simulink model "PMLSM_MIL_Library_Sim"  (R2023b)
settings: Solver=FixedStepDiscrete  StartTime=0.0  StopTime=1.5  FixedStep=1e-4  RelTol=1e-3
values from neighbouring files (symbols this model uses):
  PMLSM_grating_resolution_mm = 0.0001    [init_PMLSM_plant_params.m]
  PMLSM_Kf_N_per_A = PMLSM_Kf_peak_N_per_Apeak    [init_PMLSM_plant_params.m]
  PMLSM_Ld_H = Ld    (= 0.001745)    [PMSLM_Init_Params_MBDL4.m]    (also in init_PMLSM_plant_params.m)
  PMLSM_Lq_H = Lq    (= 0.001745)    [PMSLM_Init_Params_MBDL4.m]    (also in init_PMLSM_plant_params.m)
  PMLSM_mass_kg = PMLSM_M_kg    (= 0.91)    [init_PMLSM_plant_params.m]
  PMLSM_psi_f_Wb = flux    (= 0.141)    [PMSLM_Init_Params_MBDL4.m]    (also in init_PMLSM_plant_params.m)
  PMLSM_pwm_period_counts = 7500    [init_PMLSM_plant_params.m]
  PMLSM_Rs_ohm = Rs    (= 2.37)    [PMSLM_Init_Params_MBDL4.m]    (also in init_PMLSM_plant_params.m)
  PMLSM_sensor_delay_samples = 50    [init_PMLSM_plant_params.m]
  PMLSM_tau_e_mm = PMLSM_tau_NN_mm    (= 60)    [init_PMLSM_plant_params.m]
  PMLSM_theta_offset_rad = 0    [init_PMLSM_plant_params.m]
  PMLSM_Ts_s = 1e-4    (= 0.0001)    [init_PMLSM_plant_params.m]
  PMLSM_vdc_V = 48    [init_PMLSM_plant_params.m]
  PMLSM_viscous_N_per_mps = PMLSM_Bv_N_per_mps    (= 0)    [init_PMLSM_plant_params.m]
undefined symbols (not defined in the file or in its folder): DiscIntNeverNeededParam
settings Model: Creator=lww  LastModifiedBy=lww

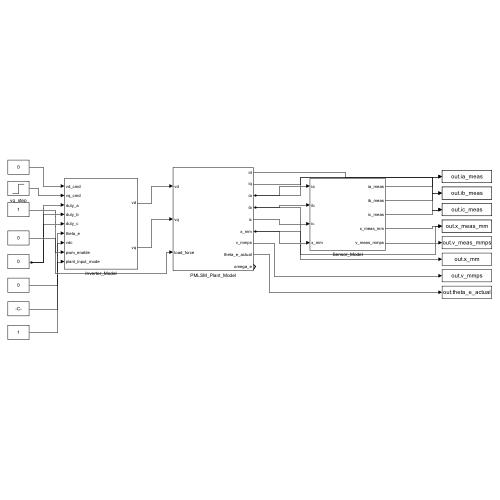
[thumbnail: Simulink's stored preview of the top-level diagram]
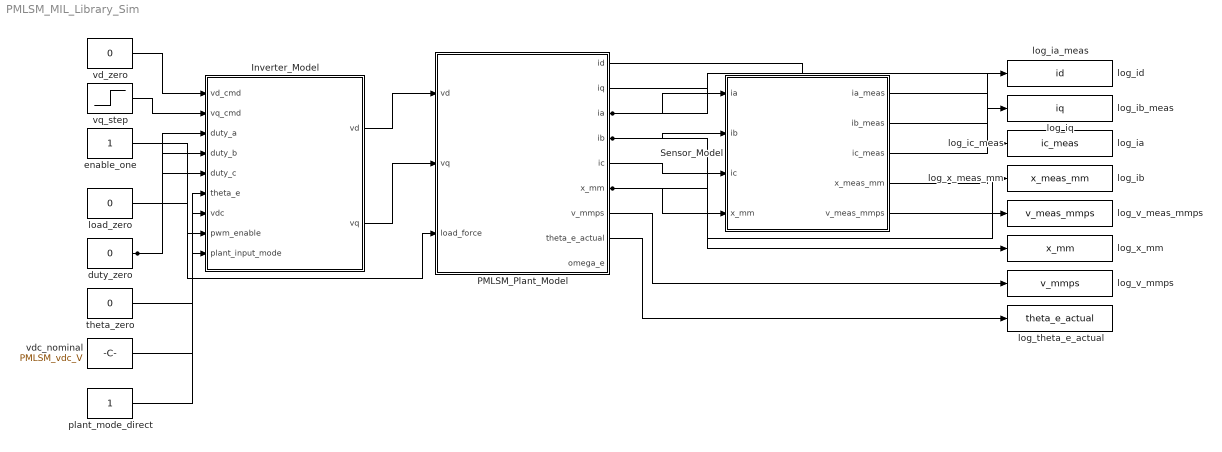
== system PMLSM_MIL_Library_Sim ==
  Inverter_Model : Subsystem
  PMLSM_Plant_Model : Subsystem
  Sensor_Model : Subsystem
  duty_zero : Constant  Value=0
  enable_one : Constant
  load_zero : Constant  Value=0
  log_ia : ToWorkspace  VariableName=ia  SaveFormat=Timeseries  SampleTime=-1
  log_ia_meas : ToWorkspace  VariableName=ia_meas  SaveFormat=Timeseries  SampleTime=-1
  log_ib : ToWorkspace  VariableName=ib  SaveFormat=Timeseries  SampleTime=-1
  log_ib_meas : ToWorkspace  VariableName=ib_meas  SaveFormat=Timeseries  SampleTime=-1
  log_ic_meas : ToWorkspace  VariableName=ic_meas  SaveFormat=Timeseries  SampleTime=-1
  log_id : ToWorkspace  VariableName=id  SaveFormat=Timeseries  SampleTime=-1
  log_iq : ToWorkspace  VariableName=iq  SaveFormat=Timeseries  SampleTime=-1
  log_theta_e_actual : ToWorkspace  VariableName=theta_e_actual  SaveFormat=Timeseries  SampleTime=-1
  log_v_meas_mmps : ToWorkspace  VariableName=v_meas_mmps  SaveFormat=Timeseries  SampleTime=-1
  log_v_mmps : ToWorkspace  VariableName=v_mmps  SaveFormat=Timeseries  SampleTime=-1
  log_x_meas_mm : ToWorkspace  VariableName=x_meas_mm  SaveFormat=Timeseries  SampleTime=-1
  log_x_mm : ToWorkspace  VariableName=x_mm  SaveFormat=Timeseries  SampleTime=-1
  plant_mode_direct : Constant
  theta_zero : Constant  Value=0
  vd_zero : Constant  Value=0
  vdc_nominal : Constant  Value=PMLSM_vdc_V
  vq_step : Step  Time=0.05  After=0.8  SampleTime=0
  wires:
  vd_zero/1 -> Inverter_Model/1(vd_cmd)
  vq_step/1 -> Inverter_Model/2(vq_cmd)
  duty_zero/1 -> Inverter_Model/3(duty_a), Inverter_Model/4(duty_b), Inverter_Model/5(duty_c)
  theta_zero/1 -> Inverter_Model/6(theta_e)
  vdc_nominal/1 -> Inverter_Model/7(vdc)
  enable_one/1 -> Inverter_Model/8(pwm_enable)
  plant_mode_direct/1 -> Inverter_Model/9(plant_input_mode)
  Inverter_Model/1(vd) -> PMLSM_Plant_Model/1(vd)
  Inverter_Model/2(vq) -> PMLSM_Plant_Model/2(vq)
  load_zero/1 -> PMLSM_Plant_Model/3(load_force)
  PMLSM_Plant_Model/3(ia) -> Sensor_Model/1(ia), log_ia/1
  PMLSM_Plant_Model/4(ib) -> Sensor_Model/2(ib), log_ib/1
  PMLSM_Plant_Model/5(ic) -> Sensor_Model/3(ic)
  PMLSM_Plant_Model/6(x_mm) -> Sensor_Model/4(x_mm), log_x_mm/1
  PMLSM_Plant_Model/1(id) -> log_id/1
  PMLSM_Plant_Model/2(iq) -> log_iq/1
  PMLSM_Plant_Model/7(v_mmps) -> log_v_mmps/1
  PMLSM_Plant_Model/8(theta_e_actual) -> log_theta_e_actual/1
  Sensor_Model/1(ia_meas) -> log_ia_meas/1
  Sensor_Model/2(ib_meas) -> log_ib_meas/1
  Sensor_Model/3(ic_meas) -> log_ic_meas/1
  Sensor_Model/4(x_meas_mm) -> log_x_meas_mm/1
  Sensor_Model/5(v_meas_mmps) -> log_v_meas_mmps/1

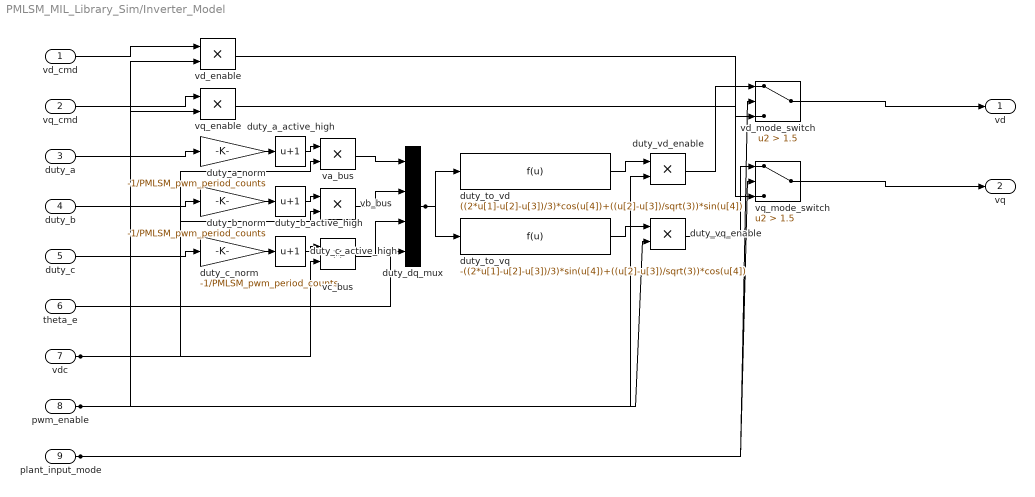
== system PMLSM_MIL_Library_Sim/Inverter_Model ==
  vd_cmd : Inport
  vq_cmd : Inport  Port=2
  duty_a : Inport  Port=3
  duty_b : Inport  Port=4
  duty_c : Inport  Port=5
  theta_e : Inport  Port=6
  vdc : Inport  Port=7
  pwm_enable : Inport  Port=8
  plant_input_mode : Inport  Port=9
  duty_a_active_high : Bias  Bias=1  SaturateOnIntegerOverflow=off
  duty_a_norm : Gain  Gain=-1/PMLSM_pwm_period_counts
  duty_b_active_high : Bias  Bias=1  SaturateOnIntegerOverflow=off
  duty_b_norm : Gain  Gain=-1/PMLSM_pwm_period_counts
  duty_c_active_high : Bias  Bias=1  SaturateOnIntegerOverflow=off
  duty_c_norm : Gain  Gain=-1/PMLSM_pwm_period_counts
  duty_dq_mux : Mux
  duty_to_vd : Fcn  Expr=((2*u[1]-u[2]-u[3])/3)*cos(u[4])+((u[2]-u[3])/sqrt(3))*sin(u[4])
  duty_to_vq : Fcn  Expr=-((2*u[1]-u[2]-u[3])/3)*sin(u[4])+((u[2]-u[3])/sqrt(3))*cos(u[4])
  duty_vd_enable : Product
  duty_vq_enable : Product
  va_bus : Product
  vb_bus : Product
  vc_bus : Product
  vd_enable : Product
  vd_mode_switch : Switch  Criteria=u2 > Threshold  Threshold=1.5  SaturateOnIntegerOverflow=off  InputSameDT=off
  vq_enable : Product
  vq_mode_switch : Switch  Criteria=u2 > Threshold  Threshold=1.5  SaturateOnIntegerOverflow=off  InputSameDT=off
  vd : Outport
  vq : Outport  Port=2
  wires:
  ? -> ?
  vd_cmd/1 -> vd_enable/1
  pwm_enable/1 -> vd_enable/2, vq_enable/2, duty_vd_enable/2, duty_vq_enable/2
  vq_cmd/1 -> vq_enable/1
  duty_a/1 -> duty_a_norm/1
  duty_b/1 -> duty_b_norm/1
  duty_c/1 -> duty_c_norm/1
  duty_a_norm/1 -> duty_a_active_high/1
  duty_b_norm/1 -> duty_b_active_high/1
  duty_c_norm/1 -> duty_c_active_high/1
  duty_a_active_high/1 -> va_bus/1
  duty_b_active_high/1 -> vb_bus/1
  duty_c_active_high/1 -> vc_bus/1
  vdc/1 -> va_bus/2, vb_bus/2, vc_bus/2
  va_bus/1 -> duty_dq_mux/1
  vb_bus/1 -> duty_dq_mux/2
  vc_bus/1 -> duty_dq_mux/3
  theta_e/1 -> duty_dq_mux/4
  duty_dq_mux/1 -> duty_to_vd/1, duty_to_vq/1
  duty_to_vd/1 -> duty_vd_enable/1
  duty_to_vq/1 -> duty_vq_enable/1
  duty_vd_enable/1 -> vd_mode_switch/1
  plant_input_mode/1 -> vd_mode_switch/2, vq_mode_switch/2
  vd_enable/1 -> vd_mode_switch/3
  duty_vq_enable/1 -> vq_mode_switch/1
  vq_enable/1 -> vq_mode_switch/3
  vd_mode_switch/1 -> vd/1
  vq_mode_switch/1 -> vq/1

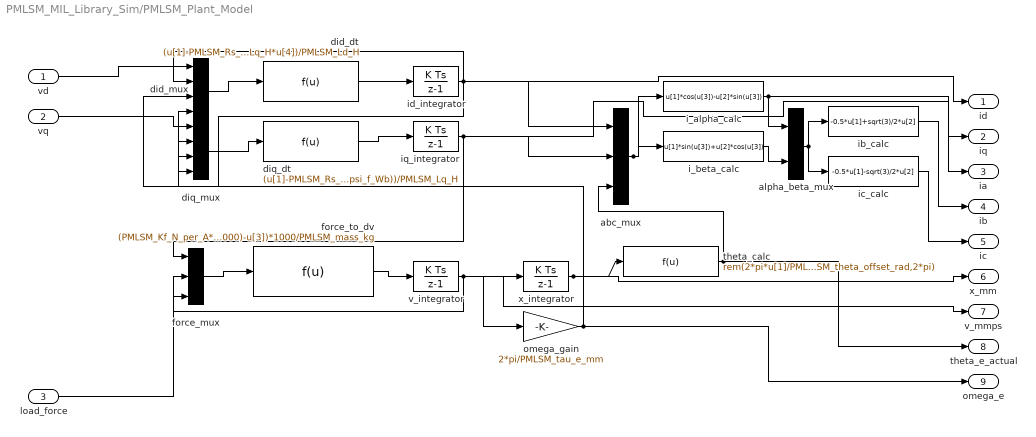
== system PMLSM_MIL_Library_Sim/PMLSM_Plant_Model ==
  vd : Inport
  vq : Inport  Port=2
  load_force : Inport  Port=3
  abc_mux : Mux  Inputs=3
  alpha_beta_mux : Mux  Inputs=2
  did_dt : Fcn  Expr=(u[1]-PMLSM_Rs_ohm*u[2]+u[3]*PMLSM_Lq_H*u[4])/PMLSM_Ld_H
  did_mux : Mux
  diq_dt : Fcn  Expr=(u[1]-PMLSM_Rs_ohm*u[2]-u[3]*(PMLSM_Ld_H*u[4]+PMLSM_psi_f_Wb))/PMLSM_Lq_H
  diq_mux : Mux
  force_mux : Mux  Inputs=3
  force_to_dv : Fcn  Expr=(PMLSM_Kf_N_per_A*u[1]-PMLSM_viscous_N_per_mps*(u[2]/1000)-u[3])*1000/PMLSM_mass_kg
  i_alpha_calc : Fcn  Expr=u[1]*cos(u[3])-u[2]*sin(u[3])
  i_beta_calc : Fcn  Expr=u[1]*sin(u[3])+u[2]*cos(u[3])
  ib_calc : Fcn  Expr=-0.5*u[1]+sqrt(3)/2*u[2]
  ic_calc : Fcn  Expr=-0.5*u[1]-sqrt(3)/2*u[2]
  id_integrator : DiscreteIntegrator  gainval=1  SampleTime=PMLSM_Ts_s  ICPrevOutput=DiscIntNeverNeededParam  ICPrevScaledInput=DiscIntNeverNeededParam
  iq_integrator : DiscreteIntegrator  gainval=1  SampleTime=PMLSM_Ts_s  ICPrevOutput=DiscIntNeverNeededParam  ICPrevScaledInput=DiscIntNeverNeededParam
  omega_gain : Gain  Gain=2*pi/PMLSM_tau_e_mm
  theta_calc : Fcn  Expr=rem(2*pi*u[1]/PMLSM_tau_e_mm+PMLSM_theta_offset_rad,2*pi)
  v_integrator : DiscreteIntegrator  gainval=1  SampleTime=PMLSM_Ts_s  ICPrevOutput=DiscIntNeverNeededParam  ICPrevScaledInput=DiscIntNeverNeededParam
  x_integrator : DiscreteIntegrator  gainval=1  SampleTime=PMLSM_Ts_s  ICPrevOutput=DiscIntNeverNeededParam  ICPrevScaledInput=DiscIntNeverNeededParam
  id : Outport
  iq : Outport  Port=2
  ia : Outport  Port=3
  ib : Outport  Port=4
  ic : Outport  Port=5
  x_mm : Outport  Port=6
  v_mmps : Outport  Port=7
  theta_e_actual : Outport  Port=8
  omega_e : Outport  Port=9
  wires:
  ? -> ?
  vd/1 -> did_mux/1
  id_integrator/1 -> did_mux/2, diq_mux/4, abc_mux/1, id/1
  omega_gain/1 -> did_mux/3, diq_mux/3, omega_e/1
  iq_integrator/1 -> did_mux/4, diq_mux/2, force_mux/1, abc_mux/2, iq/1
  did_mux/1 -> did_dt/1
  did_dt/1 -> id_integrator/1
  vq/1 -> diq_mux/1
  diq_mux/1 -> diq_dt/1
  diq_dt/1 -> iq_integrator/1
  v_integrator/1 -> force_mux/2, x_integrator/1, omega_gain/1, v_mmps/1
  load_force/1 -> force_mux/3
  force_mux/1 -> force_to_dv/1
  force_to_dv/1 -> v_integrator/1
  x_integrator/1 -> theta_calc/1, x_mm/1
  theta_calc/1 -> abc_mux/3, theta_e_actual/1
  abc_mux/1 -> i_alpha_calc/1, i_beta_calc/1
  i_alpha_calc/1 -> alpha_beta_mux/1, ia/1
  i_beta_calc/1 -> alpha_beta_mux/2
  alpha_beta_mux/1 -> ib_calc/1, ic_calc/1
  ib_calc/1 -> ib/1
  ic_calc/1 -> ic/1

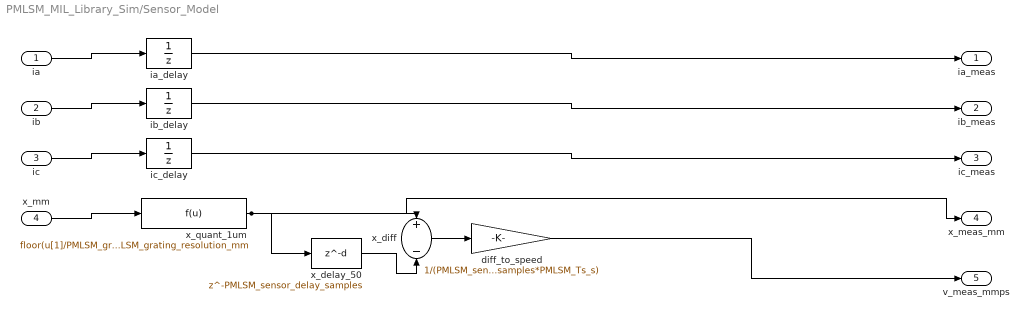
== system PMLSM_MIL_Library_Sim/Sensor_Model ==
  ia : Inport
  ib : Inport  Port=2
  ic : Inport  Port=3
  x_mm : Inport  Port=4
  diff_to_speed : Gain  Gain=1/(PMLSM_sensor_delay_samples*PMLSM_Ts_s)
  ia_delay : UnitDelay  SampleTime=PMLSM_Ts_s  HasFrameUpgradeWarning=on
  ib_delay : UnitDelay  SampleTime=PMLSM_Ts_s  HasFrameUpgradeWarning=on
  ic_delay : UnitDelay  SampleTime=PMLSM_Ts_s  HasFrameUpgradeWarning=on
  x_delay_50 : Delay  DelayLength=PMLSM_sensor_delay_samples  InitialCondition=0  SampleTime=PMLSM_Ts_s
  x_diff : Sum  Inputs=+-
  x_quant_1um : Fcn  Expr=floor(u[1]/PMLSM_grating_resolution_mm+0.5)*PMLSM_grating_resolution_mm
  ia_meas : Outport
  ib_meas : Outport  Port=2
  ic_meas : Outport  Port=3
  x_meas_mm : Outport  Port=4
  v_meas_mmps : Outport  Port=5
  wires:
  ? -> ?
  ia/1 -> ia_delay/1
  ib/1 -> ib_delay/1
  ic/1 -> ic_delay/1
  x_mm/1 -> x_quant_1um/1
  x_quant_1um/1 -> x_delay_50/1, x_diff/1, x_meas_mm/1
  x_delay_50/1 -> x_diff/2
  x_diff/1 -> diff_to_speed/1
  ia_delay/1 -> ia_meas/1
  ib_delay/1 -> ib_meas/1
  ic_delay/1 -> ic_meas/1
  diff_to_speed/1 -> v_meas_mmps/1
